simulink model "quart_vehicule"  (R2026a)
settings: Solver=FixedStepAuto  StopTime=10  FixedStep=1e-3
values from neighbouring files (symbols this model uses):
  b1 = 87.5    [Automotive_suspension_parameters.m]    (also in parametres_suspension.m)
  b2 = 3755    [Automotive_suspension_parameters.m]    (also in parametres_suspension.m)
  k1 = 20000    [Automotive_suspension_parameters.m]    (also in parametres_suspension.m)
  k2 = 125000    [Automotive_suspension_parameters.m]    (also in parametres_suspension.m)
  m1 = 500    [Automotive_suspension_parameters.m]    (also in parametres_suspension.m)
  m2 = 80    [Automotive_suspension_parameters.m]    (also in parametres_suspension.m)
libraries: slpidlib x1, simulink x1
settings Model: Creator=Moi  LastModifiedBy=lulu1

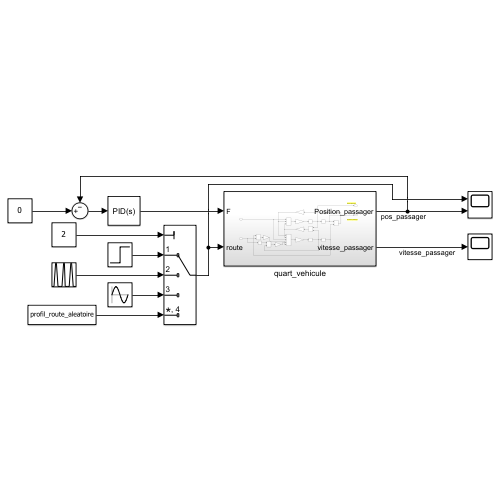
[thumbnail: Simulink's stored preview of the top-level diagram]
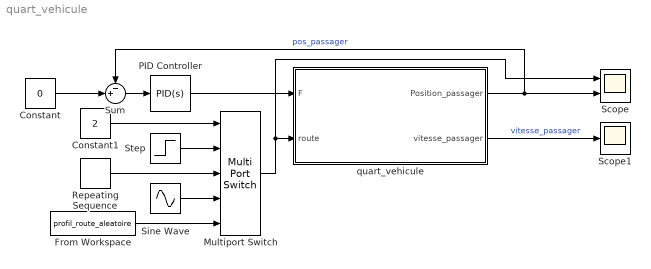
== system quart_vehicule ==
  Constant : Constant  Value=0
  Constant1 : Constant  Value=2
  From Workspace : FromWorkspace  VariableName=profil_route_aleatoire  SampleTime=1/1000  OutputAfterFinalValue=Setting to zero
  Multiport Switch : MultiPortSwitch  Inputs=4  SaturateOnIntegerOverflow=off  InputSameDT=off
  PID Controller : slpidlib/PID Controller  Controller=PID  Form=Parallel  TimeDomain=Continuous-time  UseExternalTs=off  SampleTime=-1  IntegratorMethod=Forward Euler  FilterMethod=Forward Euler  ControllerParametersSource=internal  P=16718739.2087504  I=335534728.670535  UseKiTs=off  D=204621.50544303  UseExternalDerivativeSource=off  N=2296.86311935817  UseFilter=on  TunerSelectOption=Transfer Function Based (PID Tuner App)  InitialConditionSource=internal  InitialConditionForIntegrator=0  InitialConditionForFilter=0  DifferentiatorICPrevScaledInput=0  ExternalReset=none  TrackingMode=off  Kt=1  LimitOutput=off  SatLimitsSource=internal  UpperSaturationLimit=inf  LowerSaturationLimit=-inf  LinearizeAsGain=on  AntiWindupMode=none  Kb=1  LimitIntegrator=off  UpperIntegratorSaturationLimit=inf  LowerIntegratorSaturationLimit=-inf  POutMin=[]  POutMax=[]  IOutMin=[]  IOutMax=[]  DOutMin=[]  DOutMax=[]  NOutMin=[]  NOutMax=[]  SumOutMin=[]  SumOutMax=[]  SaturationOutMin=[]  SaturationOutMax=[]  PParamMin=[]  PParamMax=[]  IParamMin=[]  IParamMax=[]  DParamMin=[]  DParamMax=[]  NParamMin=[]  NParamMax=[]  KbParamMin=[]  KbParamMax=[]  KtParamMin=[]  KtParamMax=[]  KbOutMin=[]  KbOutMax=[]  KtOutMin=[]  KtOutMax=[]  IntegratorOutMin=[]  IntegratorOutMax=[]  FilterOutMin=[]  FilterOutMax=[]  SumI1OutMin=[]  SumI1OutMax=[]  SumI2OutMin=[]  SumI2OutMax=[]  SumI3OutMin=[]  SumI3OutMax=[]  SumI4OutMin=[]  SumI4OutMax=[]  SumDOutMin=[]  SumDOutMax=[]  DifferentiatorOutMin=[]  DifferentiatorOutMax=[]  FilterDiffOutCoefMin=[]  FilterDiffOutCoefMax=[]  ReciprocalOutMin=[]  ReciprocalOutMax=[]  SumDenOutMin=[]  SumDenOutMax=[]  SumNumOutMin=[]  SumNumOutMax=[]  DivideOutMin=[]  DivideOutMax=[]  UdiffTsProdOutMin=[]  UdiffTsProdOutMax=[]  NTsProdOutMin=[]  NTsProdOutMax=[]  UintegralTsProdOutMin=[]  UintegralTsProdOutMax=[]  UngainTsProdOutMin=[]  UngainTsProdOutMax=[]  ClampingZeroOutDataTypeStr=Inherit: Inherit via back propagation  ClampingZeroOutMin=[]  ClampingZeroOutMax=[]  FilterDenConstantOutDataTypeStr=Inherit: Inherit via back propagation  FilterDenConstantOutMin=[]  FilterDenConstantOutMax=[]  PCopyOutDataTypeStr=Inherit: Inherit via back propagation  PCopyOutMin=[]  PCopyOutMax=[]  NCopyOutDataTypeStr=Inherit: Inherit via back propagation  NCopyOutMin=[]  NCopyOutMax=[]  IntegratorContinuousStateAttributes=''  IntegratorStateMustResolveToSignalObject=off  IntegratorRTWStateStorageClass=Auto  FilterContinuousStateAttributes=''  FilterStateMustResolveToSignalObject=off  FilterRTWStateStorageClass=Auto  ParallelPVariant=InternalParameters  IdealPVariant=Disabled  IVariant=InternalParameters  DVariant=InternalParameters  IntegratorVariant=Continuous  SatVariant=Disabled  AWVariant=Passthrough  PCopyVariant=Disabled  TRVariant=Disabled  FdbkBlocksVariant=Forward  IdealPFdbkVariant=Disabled  SatFdbkVariant=Disabled  DerivativeFilterVariant=ContFilter  NVariant=InternalParameters  NCopyVariant=Disabled  FilterICVariant=InternalICsFilter  IntegratorICVariant=InternalICs  ExternalResetVariant=Disabled  TRSumVariant=Passthrough  SumFdbkVariant=Disabled  SumVariant=Sum_PID  TsampFilterVariant=InternalTs  TsampNgainVariant=Passthrough  TsampIntegralVariant=Disabled_SignalSpec  ExternalSaturationOutDataTypeStr=Inherit: Same as second input  DerivativeSourceVariant=ErrorSignal  PreIntVariant=InternalPreInt
  Repeating Sequence : simulink/Sources/Repeating Sequence  rep_seq_t=[0 2 4 5 7 10]  rep_seq_y=[0 0 0.1 0.1 0 0]
  Scope : Scope  NumInputPorts=2
      settings: ActiveDisplayYMinimum=-0.012503581551431312  ActiveDisplayYMaximum=0.11250039795015904
  Scope1 : Scope
      settings: ActiveDisplayYMinimum=-0.25659964405144886  ActiveDisplayYMaximum=0.247946125519848
  Sine Wave : Sin  Amplitude=0.1  Frequency=2*pi*3  SampleTime=0
  Step : Step  FinalValue=0.015  SampleTime=0
  Sum : Sum  Inputs=-+|
  quart_vehicule : Subsystem
  wires:
  quart_vehicule/1(Position_passager) -> Sum/1, Scope/2  "pos_passager"
  quart_vehicule/2(vitesse_passager) -> Scope1/1  "vitesse_passager"
  Multiport Switch/1 -> Scope/1, quart_vehicule/2(route)
  Step/1 -> Multiport Switch/2
  Sine Wave/1 -> Multiport Switch/4
  Constant1/1 -> Multiport Switch/1
  Repeating Sequence/1 -> Multiport Switch/3
  From Workspace/1 -> Multiport Switch/5
  Constant/1 -> Sum/2
  PID Controller/1 -> quart_vehicule/1(F)
  Sum/1 -> PID Controller/1

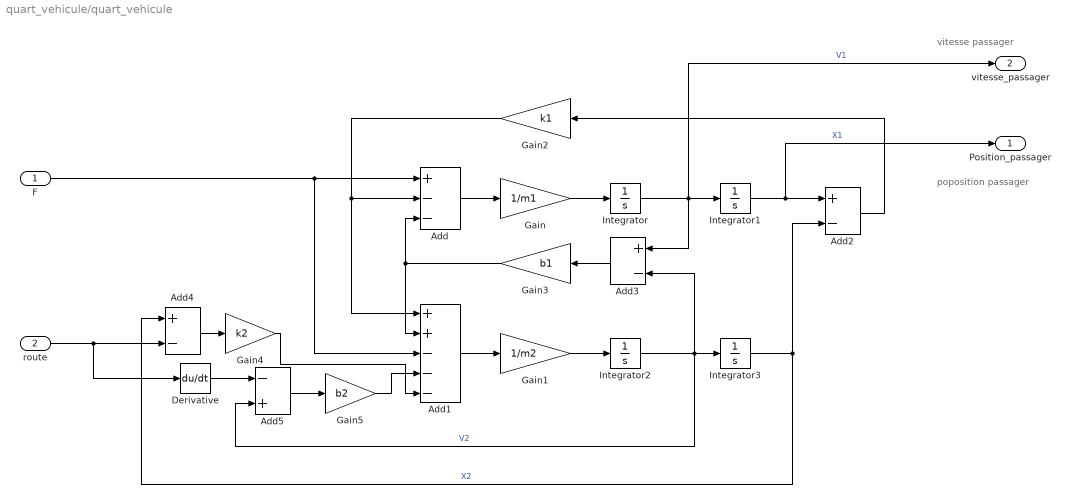
== system quart_vehicule/quart_vehicule ==
  note: vitesse passager
  note: poposition passager
  F : Inport
  route : Inport  Port=2
  Add : Sum  Inputs=+--
  Add1 : Sum  Inputs=++---
  Add2 : Sum  Inputs=+-
  Add3 : Sum  Inputs=+-
  Add4 : Sum  Inputs=+-
  Add5 : Sum  Inputs=-+
  Derivative : Derivative
  Gain : Gain  Gain=1/m1
  Gain1 : Gain  Gain=1/m2
  Gain2 : Gain  Gain=k1
  Gain3 : Gain  Gain=b1
  Gain4 : Gain  Gain=k2
  Gain5 : Gain  Gain=b2
  Integrator{,1..3} (4 alike) : Integrator
  Position_passager : Outport
  vitesse_passager : Outport  Port=2
  wires:
  Gain5/1 -> Add1/4
  Integrator1/1 -> Position_passager/1, Add2/1  "X1"
  Add1/1 -> Gain1/1
  Add/1 -> Gain/1
  F/1 -> Add/1, Add1/3
  Gain3/1 -> Add/3, Add1/2
  Integrator2/1 -> Integrator3/1, Add3/2, Add5/2  "V2"
  Add4/1 -> Gain4/1
  Derivative/1 -> Add5/1
  route/1 -> Add4/2, Derivative/1
  Add2/1 -> Gain2/1
  Add3/1 -> Gain3/1
  Integrator/1 -> vitesse_passager/1, Integrator1/1, Add3/1  "V1"
  Add5/1 -> Gain5/1
  Integrator3/1 -> Add2/2, Add4/1  "X2"
  Gain/1 -> Integrator/1
  Gain4/1 -> Add1/5
  Gain1/1 -> Integrator2/1
  Gain2/1 -> Add/2, Add1/1
